simulink model "simulink_model_closed_loop"  (R2016b)
settings: Solver=ode45  StartTime=0.0  StopTime=1  RelTol=1e-3
values from neighbouring files (symbols this model uses):
  N = 40    [extensive_example_ocp.m]    (also in minimal_example_closed_loop.m = 20; minimal_example_ocp.m = 20)
  nu = model.u.rows()    [extensive_example_ocp.m]    (also in get_pendulum_on_cart_model.m = 1; minimal_example_closed_loop.m; minimal_example_ocp.m = length(model.u))
  ny = nx+nu    [extensive_example_ocp.m]    (also in minimal_example_ocp.m = nx + nu)
  ny_0 = nu    [extensive_example_ocp.m]    (also in minimal_example_ocp.m)
  ny_e = nx    [extensive_example_ocp.m]    (also in minimal_example_ocp.m)
  U_max = 80    [minimal_example_closed_loop.m]    (also in minimal_example_ocp.m)
  x0 = [0; pi; 0; 0]    [extensive_example_ocp.m]    (also in minimal_example_closed_loop.m = x_sim(:,i); minimal_example_ocp.m; minimal_example_sim.m = [0; 1e-1; 0; 0])
settings Model: Creator=oj  LastModifiedBy=oj
settings DataIOCC: SaveFormat=StructureWithTime  ReturnWorkspaceOutputs=on
settings OptimizationCC: LifeSpan=inf
settings DebuggingCC: SFExecutionAtInitializationDiag=none
settings HardwareCC: ProdBitPerSizeT=32  ProdBitPerPtrDiffT=32  ProdWordSize=32  ProdHWDeviceType=Specified
settings ModelReferenceCC: EnableRefExpFcnMdlSchedulingChecks=off
settings SFSimCC: SimUseLocalCustomCode=on
settings RTWCC: RTWUseLocalCustomCode=on

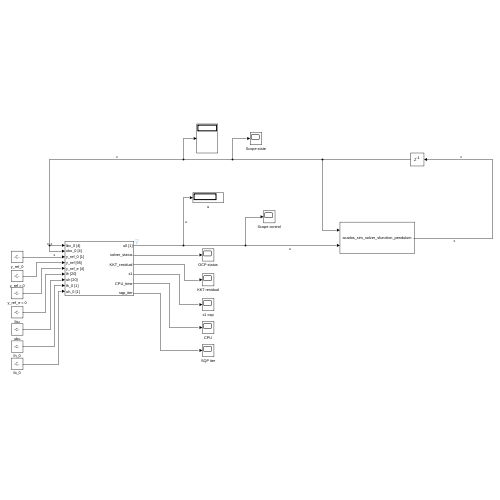
[thumbnail: Simulink's stored preview of the top-level diagram]
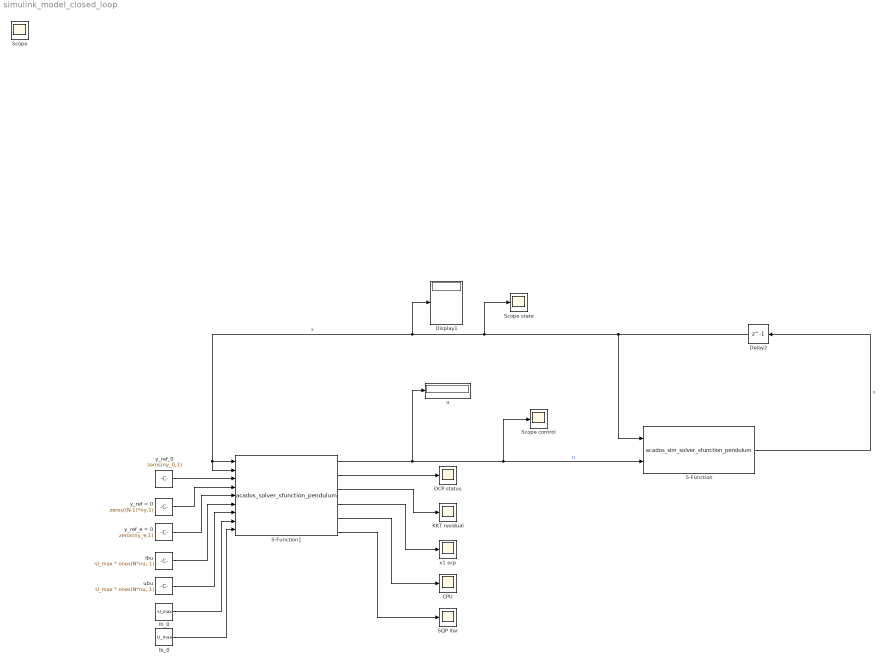
== system simulink_model_closed_loop ==
  CPU : Scope
      settings: Description=status
  Delay2 : Delay  DelayLength=1  InitialCondition=x0
  Display1 : Display
  KKT residual : Scope
      settings: Description=status
  OCP status : Scope
      settings: Description=status
  S-Function : S-Function  FunctionName=acados_sim_solver_sfunction_pendulum  SFunctionDeploymentMode=off  EnableBusSupport=off
  S-Function1 : S-Function  FunctionName=acados_solver_sfunction_pendulum  SFunctionDeploymentMode=off  EnableBusSupport=off
      mask Display:
      | % from the make_sfun file
      | global sfun_input_names sfun_output_names
      | for i = 1:length(sfun_input_names)
      | 	port_label('input', i, sfun_input_names{i})
      | end
      | for i = 1:length(sfun_output_names)
      | 	port_label('output', i, sfun_output_names{i})
      | end
  SQP iter : Scope
      settings: Description=status
  Scope control : Scope
  Scope state : Scope
  lb_0 : Constant  Value=U_max
  lbu : Constant  Value=-U_max * ones(N*nu, 1)
  lh_0 : Constant  Value=-U_max
  u : Display
  ubu : Constant  Value=U_max * ones(N*nu, 1)
  x1 ocp : Scope
      settings: Description=status
  y_ref = 0 : Constant  Value=zeros((N-1)*ny,1)
  y_ref_0 : Constant  Value=zeros(ny_0,1)
  y_ref_e = 0 : Constant  Value=zeros(ny_e,1)
  Scope : Scope
  wires:
  lb_0/1 -> S-Function1/9
  S-Function/1 -> Delay2/1  "x"
  S-Function1/1 -> u/1, Scope control/1, S-Function/2  "u"
  y_ref = 0/1 -> S-Function1/4
  ubu/1 -> S-Function1/7
  S-Function1/5 -> CPU/1
  S-Function1/6 -> SQP iter/1
  S-Function1/3 -> KKT residual/1
  Delay2/1 -> S-Function/1, S-Function1/2, S-Function1/1, Display1/1, Scope state/1  "x"
  lh_0/1 -> S-Function1/8
  lbu/1 -> S-Function1/6
  y_ref_e = 0/1 -> S-Function1/5
  S-Function1/4 -> x1 ocp/1
  S-Function1/2 -> OCP status/1
  y_ref_0/1 -> S-Function1/3
